simulink model "Sw_PMSMCtrl"  (R2025b)
settings: Solver=FixedStepDiscrete  StartTime=0.0  StopTime=10.0  RelTol=1e-3
values from neighbouring files (symbols this model uses):
  Par_Mdc_cboUdqCmd_Ovrd = 0    [Sw_PMSMCtrl.sldd]
  Par_Mdc_cfCurFc = 1000.0    [Sw_PMSMCtrl.sldd]
  Par_Mdc_cfKad = 1.0    [Sw_PMSMCtrl.sldd]
  Par_Mdc_cfKaq = 1.0    [Sw_PMSMCtrl.sldd]
  Par_Mdc_cfUdCmd = 0.0    [Sw_PMSMCtrl.sldd]
  Par_Mdc_cfUqCmd = 5.0    [Sw_PMSMCtrl.sldd]
  Par_Mtr_cfFlux = 0.0103693297    [Sw_PMSMCtrl.sldd]
  Par_Mtr_cfLd = 0.00085    [Sw_PMSMCtrl.sldd]
  Par_Mtr_cfLq = 0.00105    [Sw_PMSMCtrl.sldd]
  Par_Mtr_cfRs = 0.75    [Sw_PMSMCtrl.sldd]
  Par_Mtr_cuNp = 5    [Sw_PMSMCtrl.sldd]
  Par_Sw_cdTs = 5.0E-5    [Sw_PMSMCtrl.sldd]
libraries: Lib_PMSMCtrl x7, mcbeeMathTransformLib x3, Lib_General x2, mcbcontrolslib x1
settings Model: DataDictionary=Sw_PMSMCtrl.sldd  Creator=62555  LastModifiedBy=62555
settings SolverCC: MinimalZcImpactIntegration=on
settings OptimizationCC: DefaultParameterBehavior=Inlined  UseDivisionForNetSlopeComputation=on  GainParamInheritBuiltInType=on  UseFloatMulNetSlope=on  DefaultUnderspecifiedDataType=single  InlineInvariantSignals=on  PassReuseOutputArgsAs=Individual arguments  ZeroExternalMemoryAtStartup=off  ZeroInternalMemoryAtStartup=off  NoFixptDivByZeroProtection=on  EfficientFloat2IntCast=on  LifeSpan=1  MaxStackSize=64  OptimizeBlockOrder=speed  DifferentSizesBufferReuse=on  EfficientTunableParamExpr=on
settings DebuggingCC: SignalInfNanChecking=error  SignalRangeChecking=error  ReadBeforeWriteMsg=EnableAllAsError  WriteAfterWriteMsg=EnableAllAsError  WriteAfterReadMsg=EnableAllAsError  CheckMatrixSingularityMsg=error  IntegerOverflowMsg=error  ParameterPrecisionLossMsg=none  ParameterTunabilityLossMsg=error  UnconnectedInputMsg=error  UnconnectedOutputMsg=error  UnconnectedLineMsg=error  UniqueDataStoreMsg=error  AssertControl=DisableAll  SFUndirectedBroadcastEventsDiag=error  IntegerSaturationMsg=error  VariantConditionMismatch=error
settings HardwareCC: ProdBitPerPointer=32.0  ProdBitPerSizeT=32.0  ProdBitPerPtrDiffT=32.0  ProdLargestAtomicInteger=Long  ProdLargestAtomicFloat=Double  ProdWordSize=32.0  ProdLongLongMode=on  ProdHWDeviceType=ARM Compatible->ARM Cortex-M
settings ModelReferenceCC: UpdateModelReferenceTargets=IfOutOfDate  ModelReferenceNumInstancesAllowed=Single
settings SFSimCC: SFSimEcho=off  CompileTimeRecursionLimit=0.0  EnableRuntimeRecursion=off  MATLABDynamicMemAlloc=off
settings RTWCC: SystemTargetFile=ert.tlc  GenCodeOnly=on  TemplateMakefile=ert_default_tmf  GenerateReport=on  Toolchain=MinGW64 | gmake (64-bit Windows)  LaunchReport=on  GPUComputeCapability=3.5  Description=Embedded Coder
settings CodeAppCC: ForceParamTrailComments=on  IgnoreCustomStorageClasses=off  IgnoreTestpoints=on  OperatorAnnotations=on  SimulinkDataObjDesc=on  SFDataObjDesc=on  CustomSymbolStrGlobalVar=rt$N$M  CustomSymbolStrType=$N$M  CustomSymbolStrFcn=$N$M$F  CustomSymbolStrMacro=$N$M  InsertBlockDesc=on
settings ERTTargetCC: ExtModeTransport=3.0  ExtModeStaticAlloc=on  ExtModeStaticAllocSize=2048.0  ExtModeMexFile=ext_xcp  ExtModeIntrfLevel=Level2 - Open  ERTCustomFileTemplate=example_file_process.tlc  SuppressUnreachableDefaultCases=off  EnableSignedLeftShifts=off  EnableSignedRightShifts=off  DynamicArrayContainerType=coder::array  TargetLangStandard=C99 (ISO)  UtilityFuncGeneration=Shared location  IncludeMdlTerminateFcn=off  CombineSignalStateStructs=on  SupportAbsoluteTime=off  SubcomponentCodeInterfacePackaging=Nonreusable function  SupportComplex=off  SupportNonInlinedSFcns=on  ParenthesesLevel=Standards  CastingMode=Standards  GenerateSharedConstants=off

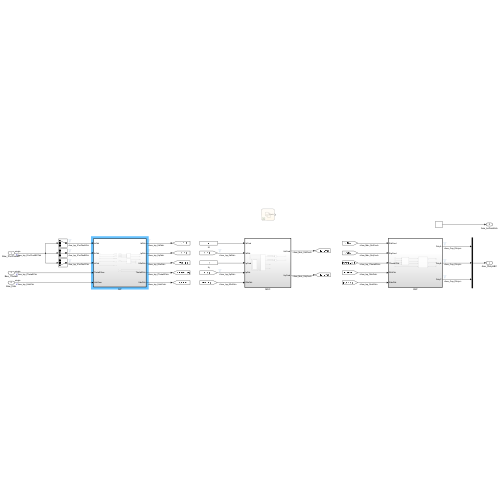
[thumbnail: Simulink's stored preview of the top-level diagram]
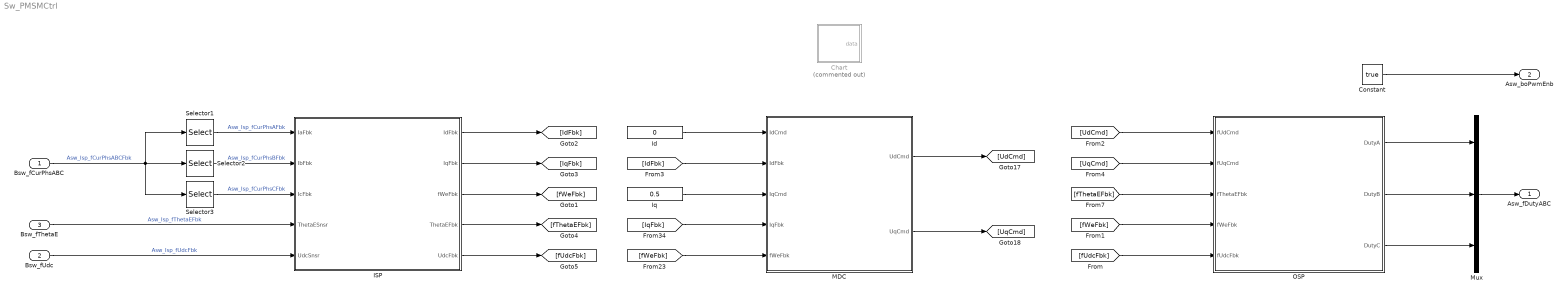
== system Sw_PMSMCtrl ==
  Bsw_fCurPhsABC : Inport  OutDataTypeStr=single  PortDimensions=3  SampleTime=Par_Sw_cdTs
  Bsw_fUdc : Inport  Port=2  OutDataTypeStr=single  SampleTime=Par_Sw_cdTs
  Bsw_fThetaE : Inport  Port=3  OutDataTypeStr=single  SampleTime=Par_Sw_cdTs
  Chart : Stateflow chart  Commented=on  TreatAsAtomicUnit=on
  Constant : Constant  Value=true  OutDataTypeStr=boolean  SampleTime=-1
  ISP : Subsystem  TreatAsAtomicUnit=on  RTWFileName=Asw_ISP
      settings: RTWSystemCode=Nonreusable function  RTWFcnNameOpts=Use subsystem name  RTWFileNameOpts=User specified  FunctionInterfaceSpec=Allow arguments (Optimized)
  Id : Constant  Value=0  OutDataTypeStr=single  SampleTime=-1
  Iq : Constant  Value=0.5  OutDataTypeStr=single  SampleTime=-1
  MDC : Subsystem  TreatAsAtomicUnit=on  RTWFileName=Asw_CLC
      settings: RTWSystemCode=Nonreusable function  RTWFcnNameOpts=Use subsystem name  RTWFileNameOpts=User specified  FunctionInterfaceSpec=Allow arguments (Optimized)
  Mux : Mux  Inputs=3
  OSP : Subsystem  TreatAsAtomicUnit=on  RTWFileName=Asw_Osp
      settings: RTWSystemCode=Nonreusable function  RTWFcnNameOpts=Use subsystem name  RTWFileNameOpts=User specified  FunctionInterfaceSpec=Allow arguments (Optimized)
  Selector1 : Selector  InputPortWidth=3  IndexOptions=Index vector (dialog)  Indices=[1]  OutputSizes=1
  Selector2 : Selector  InputPortWidth=3  IndexOptions=Index vector (dialog)  Indices=[2]  OutputSizes=1
  Selector3 : Selector  InputPortWidth=3  IndexOptions=Index vector (dialog)  Indices=[3]  OutputSizes=1
  Asw_fDutyABC : Outport
  Asw_boPwmEnb : Outport  Port=2
  wires:
  Selector1/1 -> ISP/1(IaFbk)  "Asw_Isp_fCurPhsAFbk"
  Selector2/1 -> ISP/2(IbFbk)  "Asw_Isp_fCurPhsBFbk"
  Selector3/1 -> ISP/3(IcFbk)  "Asw_Isp_fCurPhsCFbk"
  Bsw_fThetaE/1 -> ISP/4(ThetaESnsr)  "Asw_Isp_fThetaEFbk"
  Bsw_fUdc/1 -> ISP/5(UdcSnsr)  "Asw_Isp_fUdcFbk"
  ISP/1(IdFbk) -> [IdFbk]
  ISP/2(IqFbk) -> [IqFbk]
  ISP/3(fWeFbk) -> [fWeFbk]
  ISP/4(ThetaEFbk) -> [fThetaEFbk]
  ISP/5(UdcFbk) -> [fUdcFbk]
  Id/1 -> MDC/1(IdCmd)
  [IdFbk] -> MDC/2(IdFbk)
  Iq/1 -> MDC/3(IqCmd)
  [IqFbk] -> MDC/4(IqFbk)
  [fWeFbk] -> MDC/5(fWeFbk)
  MDC/1(UdCmd) -> [UdCmd]
  MDC/2(UqCmd) -> [UqCmd]
  [UdCmd] -> OSP/1(fUdCmd)
  [UqCmd] -> OSP/2(fUqCmd)
  [fThetaEFbk] -> OSP/3(fThetaEFbk)
  [fWeFbk] -> OSP/4(fWeFbk)
  [fUdcFbk] -> OSP/5(fUdcFbk)
  Constant/1 -> Asw_boPwmEnb/1
  OSP/1(DutyA) -> Mux/1
  OSP/2(DutyB) -> Mux/2
  OSP/3(DutyC) -> Mux/3
  Mux/1 -> Asw_fDutyABC/1
  Bsw_fCurPhsABC/1 -> Selector3/1, Selector2/1, Selector1/1  "Asw_Isp_fCurPhsABCFbk"

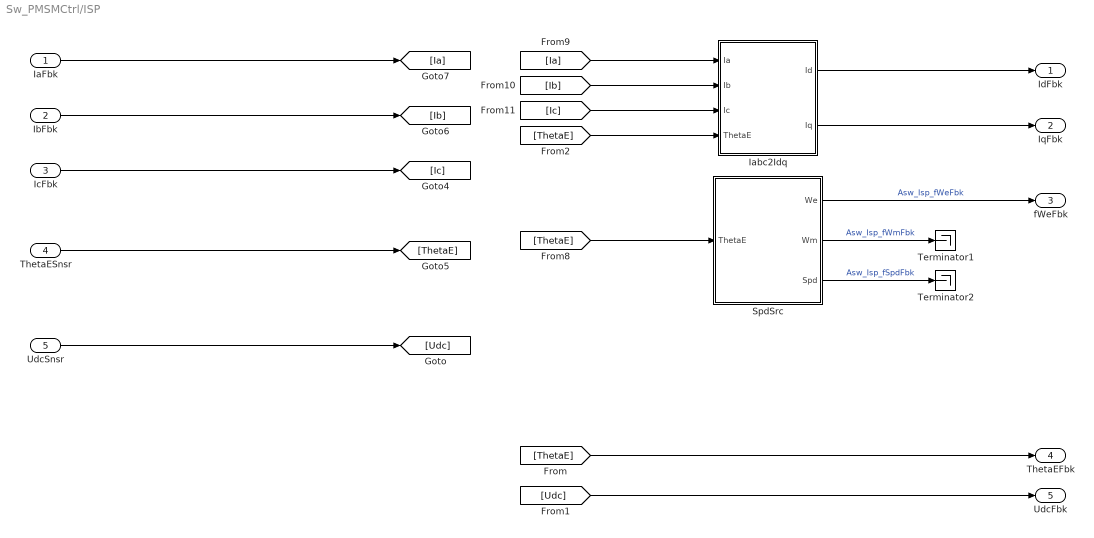
== system Sw_PMSMCtrl/ISP ==
  IaFbk : Inport
  IbFbk : Inport  Port=2
  IcFbk : Inport  Port=3
  ThetaESnsr : Inport  Port=4
  UdcSnsr : Inport  Port=5
  Iabc2Idq : Subsystem  TreatAsAtomicUnit=on
      settings: RTWSystemCode=Nonreusable function  RTWFcnNameOpts=Use subsystem name  FunctionInterfaceSpec=Allow arguments (Optimized)
  SpdSrc : Subsystem  TreatAsAtomicUnit=on
      settings: RTWSystemCode=Nonreusable function  RTWFcnNameOpts=Use subsystem name  FunctionInterfaceSpec=Allow arguments (Optimized)
  Terminator1 : Terminator
  Terminator2 : Terminator
  IdFbk : Outport
  IqFbk : Outport  Port=2
  fWeFbk : Outport  Port=3
  ThetaEFbk : Outport  Port=4
  UdcFbk : Outport  Port=5
  wires:
  SpdSrc/2(Wm) -> Terminator1/1  "Asw_Isp_fWmFbk"
  SpdSrc/3(Spd) -> Terminator2/1  "Asw_Isp_fSpdFbk"
  [ThetaE] -> Iabc2Idq/4(ThetaE)
  UdcSnsr/1 -> [Udc]
  [Ib] -> Iabc2Idq/2(Ib)
  Iabc2Idq/1(Id) -> IdFbk/1
  [ThetaE] -> SpdSrc/1(ThetaE)
  ThetaESnsr/1 -> [ThetaE]
  IcFbk/1 -> [Ic]
  IbFbk/1 -> [Ib]
  [Ia] -> Iabc2Idq/1(Ia)
  [Ic] -> Iabc2Idq/3(Ic)
  IaFbk/1 -> [Ia]
  SpdSrc/1(We) -> fWeFbk/1  "Asw_Isp_fWeFbk"
  Iabc2Idq/2(Iq) -> IqFbk/1
  [ThetaE] -> ThetaEFbk/1
  [Udc] -> UdcFbk/1

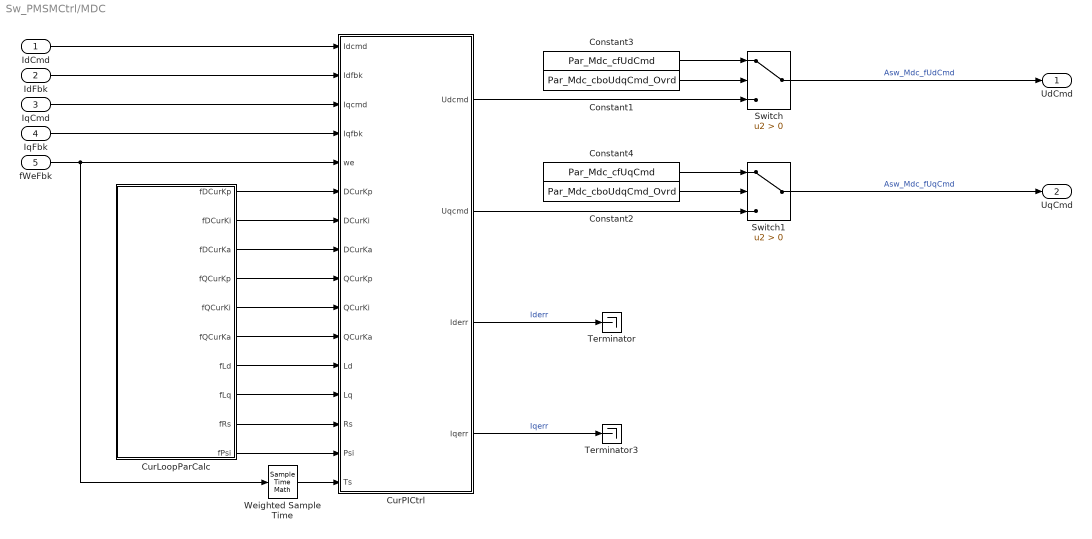
== system Sw_PMSMCtrl/MDC ==
  IdCmd : Inport
  IdFbk : Inport  Port=2
  IqCmd : Inport  Port=3
  IqFbk : Inport  Port=4
  fWeFbk : Inport  Port=5
  Constant1 : Constant  Value=Par_Mdc_cboUdqCmd_Ovrd  OutDataTypeStr=boolean  SampleTime=-1
  Constant2 : Constant  Value=Par_Mdc_cboUdqCmd_Ovrd  OutDataTypeStr=boolean  SampleTime=-1
  Constant3 : Constant  Value=Par_Mdc_cfUdCmd  OutDataTypeStr=single  SampleTime=-1
  Constant4 : Constant  Value=Par_Mdc_cfUqCmd  OutDataTypeStr=single  SampleTime=-1
  CurLoopParCalc : Subsystem
  CurPICtrl : MATLAB Function  TreatAsAtomicUnit=on
      settings: RTWSystemCode=Nonreusable function  RTWFcnNameOpts=Use subsystem name  FunctionInterfaceSpec=Allow arguments (Optimized)
  Switch : Switch  Criteria=u2 > Threshold  SaturateOnIntegerOverflow=off  InputSameDT=off
  Switch1 : Switch  Criteria=u2 > Threshold  SaturateOnIntegerOverflow=off  InputSameDT=off
  Terminator : Terminator
  Terminator3 : Terminator
  Weighted Sample Time : SampleTimeMath  TsampMathOp=Ts Only
  UdCmd : Outport
  UqCmd : Outport  Port=2
  wires:
  CurPICtrl/2(Uqcmd) -> Switch1/3
  CurPICtrl/3(Iderr) -> Terminator/1  "Iderr"
  IqCmd/1 -> CurPICtrl/3(Iqcmd)
  fWeFbk/1 -> Weighted Sample Time/1, CurPICtrl/5(we)
  IdCmd/1 -> CurPICtrl/1(Idcmd)
  CurPICtrl/1(Udcmd) -> Switch/3
  Weighted Sample Time/1 -> CurPICtrl/16(Ts)
  CurPICtrl/4(Iqerr) -> Terminator3/1  "Iqerr"
  IqFbk/1 -> CurPICtrl/4(Iqfbk)
  IdFbk/1 -> CurPICtrl/2(Idfbk)
  Constant2/1 -> Switch1/2
  Switch/1 -> UdCmd/1  "Asw_Mdc_fUdCmd"
  Constant4/1 -> Switch1/1
  Constant1/1 -> Switch/2
  Constant3/1 -> Switch/1
  Switch1/1 -> UqCmd/1  "Asw_Mdc_fUqCmd"
  CurLoopParCalc/1(fDCurKp) -> CurPICtrl/6(DCurKp)
  CurLoopParCalc/2(fDCurKi) -> CurPICtrl/7(DCurKi)
  CurLoopParCalc/3(fDCurKa) -> CurPICtrl/8(DCurKa)
  CurLoopParCalc/4(fQCurKp) -> CurPICtrl/9(QCurKp)
  CurLoopParCalc/5(fQCurKi) -> CurPICtrl/10(QCurKi)
  CurLoopParCalc/6(fQCurKa) -> CurPICtrl/11(QCurKa)
  CurLoopParCalc/7(fLd) -> CurPICtrl/12(Ld)
  CurLoopParCalc/8(fLq) -> CurPICtrl/13(Lq)
  CurLoopParCalc/9(fRs) -> CurPICtrl/14(Rs)
  CurLoopParCalc/10(fPsi) -> CurPICtrl/15(Psi)

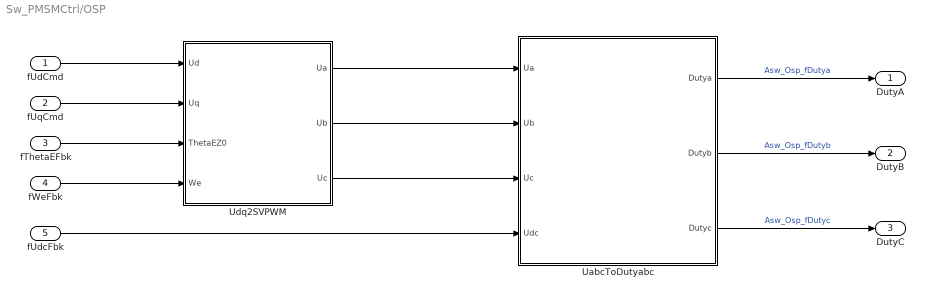
== system Sw_PMSMCtrl/OSP ==
  fUdCmd : Inport
  fUqCmd : Inport  Port=2
  fThetaEFbk : Inport  Port=3
  fWeFbk : Inport  Port=4
  fUdcFbk : Inport  Port=5
  UabcToDutyabc : Subsystem  TreatAsAtomicUnit=on
      settings: RTWSystemCode=Nonreusable function  RTWFcnNameOpts=Use subsystem name  FunctionInterfaceSpec=Allow arguments (Optimized)
  Udq2SVPWM : Subsystem  TreatAsAtomicUnit=on
      settings: RTWSystemCode=Nonreusable function  RTWFcnNameOpts=Use subsystem name  FunctionInterfaceSpec=Allow arguments (Optimized)
  DutyA : Outport
  DutyB : Outport  Port=2
  DutyC : Outport  Port=3
  wires:
  fThetaEFbk/1 -> Udq2SVPWM/3(ThetaEZ0)
  Udq2SVPWM/1(Ua) -> UabcToDutyabc/1(Ua)
  Udq2SVPWM/2(Ub) -> UabcToDutyabc/2(Ub)
  fUdCmd/1 -> Udq2SVPWM/1(Ud)
  fUdcFbk/1 -> UabcToDutyabc/4(Udc)
  Udq2SVPWM/3(Uc) -> UabcToDutyabc/3(Uc)
  fUqCmd/1 -> Udq2SVPWM/2(Uq)
  fWeFbk/1 -> Udq2SVPWM/4(We)
  UabcToDutyabc/1(Dutya) -> DutyA/1  "Asw_Osp_fDutya"
  UabcToDutyabc/2(Dutyb) -> DutyB/1  "Asw_Osp_fDutyb"
  UabcToDutyabc/3(Dutyc) -> DutyC/1  "Asw_Osp_fDutyc"

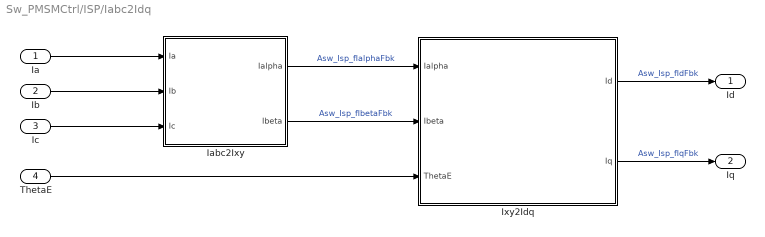
== system Sw_PMSMCtrl/ISP/Iabc2Idq ==
  Ia : Inport
  Ib : Inport  Port=2
  Ic : Inport  Port=3
  ThetaE : Inport  Port=4
  Iabc2Ixy : Subsystem  TreatAsAtomicUnit=on
      settings: RTWSystemCode=Nonreusable function  RTWFcnNameOpts=Use subsystem name  FunctionInterfaceSpec=Allow arguments (Optimized)
  Ixy2Idq : Subsystem  TreatAsAtomicUnit=on
      settings: RTWSystemCode=Nonreusable function  RTWFcnNameOpts=Use subsystem name  FunctionInterfaceSpec=Allow arguments (Optimized)
  Id : Outport
  Iq : Outport  Port=2
  wires:
  Ixy2Idq/2(Iq) -> Iq/1  "Asw_Isp_fIqFbk"
  Ia/1 -> Iabc2Ixy/1(Ia)
  ThetaE/1 -> Ixy2Idq/3(ThetaE)
  Ic/1 -> Iabc2Ixy/3(Ic)
  Ixy2Idq/1(Id) -> Id/1  "Asw_Isp_fIdFbk"
  Ib/1 -> Iabc2Ixy/2(Ib)
  Iabc2Ixy/2(Ibeta) -> Ixy2Idq/2(Ibeta)  "Asw_Isp_fIbetaFbk"
  Iabc2Ixy/1(Ialpha) -> Ixy2Idq/1(Ialpha)  "Asw_Isp_fIalphaFbk"

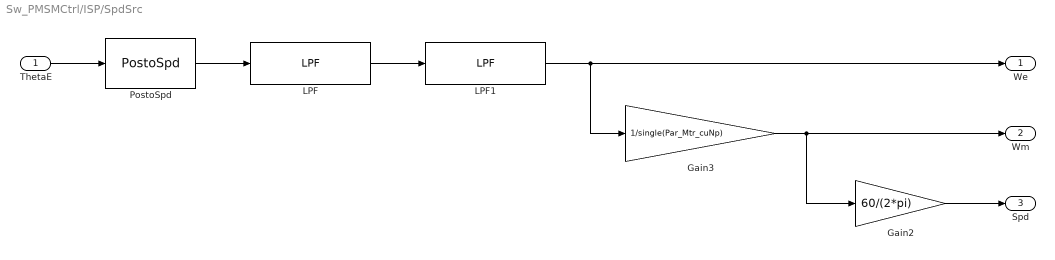
== system Sw_PMSMCtrl/ISP/SpdSrc ==
  ThetaE : Inport
  Gain2 : Gain  Gain=60/(2*pi)
  Gain3 : Gain  Gain=1/single(Par_Mtr_cuNp)
  LPF : Lib_General/LPF  fc=1e3  Initial_condition=0  ModType=Tustin
      settings: SourceProductName=Lib_General
      settings: AttributesFormatString=|
      | fc = %<fc>
      | DisMod = %<ModType>
  LPF1 : Lib_General/LPF  fc=1e3  Initial_condition=0  ModType=Tustin
      settings: SourceProductName=Lib_General
      settings: AttributesFormatString=|
      | fc = %<fc>
      | DisMod = %<ModType>
  PostoSpd : Lib_PMSMCtrl/PostoSpd
      settings: SourceProductName=Lib_PMSMCtrl
  We : Outport
  Wm : Outport  Port=2
  Spd : Outport  Port=3
  wires:
  PostoSpd/1 -> LPF/1
  ThetaE/1 -> PostoSpd/1
  Gain2/1 -> Spd/1
  Gain3/1 -> Gain2/1, Wm/1
  LPF/1 -> LPF1/1
  LPF1/1 -> We/1, Gain3/1

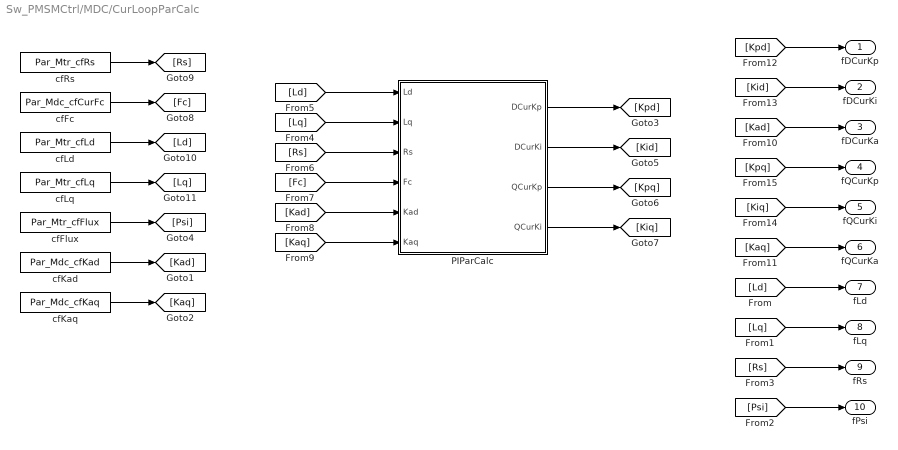
== system Sw_PMSMCtrl/MDC/CurLoopParCalc ==
  PIParCalc : MATLAB Function  TreatAsAtomicUnit=on
      settings: RTWSystemCode=Nonreusable function  RTWFcnNameOpts=Use subsystem name  FunctionInterfaceSpec=Allow arguments (Optimized)
  cfFc : Constant  Value=Par_Mdc_cfCurFc  OutDataTypeStr=single  SampleTime=-1
  cfFlux : Constant  Value=Par_Mtr_cfFlux  OutDataTypeStr=single  SampleTime=-1
  cfKad : Constant  Value=Par_Mdc_cfKad  OutDataTypeStr=single  SampleTime=-1
  cfKaq : Constant  Value=Par_Mdc_cfKaq  OutDataTypeStr=single  SampleTime=-1
  cfLd : Constant  Value=Par_Mtr_cfLd  OutDataTypeStr=single  SampleTime=-1
  cfLq : Constant  Value=Par_Mtr_cfLq  OutDataTypeStr=single  SampleTime=-1
  cfRs : Constant  Value=Par_Mtr_cfRs  OutDataTypeStr=single  SampleTime=-1
  fDCurKp : Outport
  fDCurKi : Outport  Port=2
  fDCurKa : Outport  Port=3
  fQCurKp : Outport  Port=4
  fQCurKi : Outport  Port=5
  fQCurKa : Outport  Port=6
  fLd : Outport  Port=7
  fLq : Outport  Port=8
  fRs : Outport  Port=9
  fPsi : Outport  Port=10
  wires:
  cfLq/1 -> [Lq]
  cfLd/1 -> [Ld]
  cfRs/1 -> [Rs]
  cfFc/1 -> [Fc]
  cfFlux/1 -> [Psi]
  [Ld] -> fLd/1
  [Lq] -> fLq/1
  [Psi] -> fPsi/1
  [Rs] -> fRs/1
  [Lq] -> PIParCalc/2(Lq)
  [Ld] -> PIParCalc/1(Ld)
  [Rs] -> PIParCalc/3(Rs)
  [Fc] -> PIParCalc/4(Fc)
  PIParCalc/1(DCurKp) -> [Kpd]
  cfKaq/1 -> [Kaq]
  cfKad/1 -> [Kad]
  [Kad] -> PIParCalc/5(Kad)
  [Kaq] -> PIParCalc/6(Kaq)
  [Kaq] -> fQCurKa/1
  [Kad] -> fDCurKa/1
  [Kpd] -> fDCurKp/1
  PIParCalc/2(DCurKi) -> [Kid]
  PIParCalc/3(QCurKp) -> [Kpq]
  PIParCalc/4(QCurKi) -> [Kiq]
  [Kid] -> fDCurKi/1
  [Kiq] -> fQCurKi/1
  [Kpq] -> fQCurKp/1

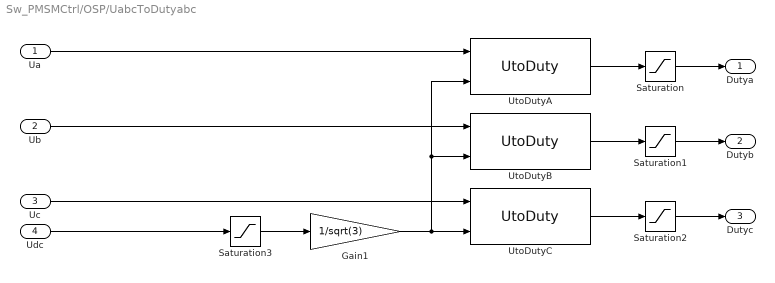
== system Sw_PMSMCtrl/OSP/UabcToDutyabc ==
  Ua : Inport
  Ub : Inport  Port=2
  Uc : Inport  Port=3
  Udc : Inport  Port=4
  Gain1 : Gain  Gain=1/sqrt(3)
  Saturation : Saturate  UpperLimit=single(1)  LowerLimit=single(0)
  Saturation1 : Saturate  UpperLimit=single(1)  LowerLimit=single(0)
  Saturation2 : Saturate  UpperLimit=single(1)  LowerLimit=single(0)
  Saturation3 : Saturate  UpperLimit=inf  LowerLimit=single(0.01)
  UtoDutyA : Lib_PMSMCtrl/UtoDuty
      settings: SourceProductName=Lib_PMSMCtrl
  UtoDutyB : Lib_PMSMCtrl/UtoDuty
      settings: SourceProductName=Lib_PMSMCtrl
  UtoDutyC : Lib_PMSMCtrl/UtoDuty
      settings: SourceProductName=Lib_PMSMCtrl
  Dutya : Outport
  Dutyb : Outport  Port=2
  Dutyc : Outport  Port=3
  wires:
  Uc/1 -> UtoDutyC/1
  Ub/1 -> UtoDutyB/1
  UtoDutyA/1 -> Saturation/1
  UtoDutyC/1 -> Saturation2/1
  UtoDutyB/1 -> Saturation1/1
  Ua/1 -> UtoDutyA/1
  Udc/1 -> Saturation3/1
  Saturation3/1 -> Gain1/1
  Gain1/1 -> UtoDutyA/2, UtoDutyB/2, UtoDutyC/2
  Saturation/1 -> Dutya/1
  Saturation1/1 -> Dutyb/1
  Saturation2/1 -> Dutyc/1

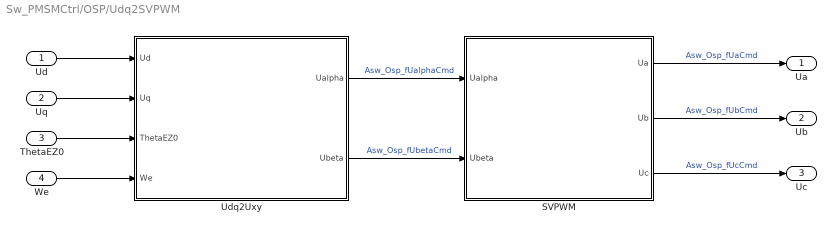
== system Sw_PMSMCtrl/OSP/Udq2SVPWM ==
  Ud : Inport
  Uq : Inport  Port=2
  ThetaEZ0 : Inport  Port=3
  We : Inport  Port=4
  SVPWM : Subsystem  TreatAsAtomicUnit=on
      settings: RTWSystemCode=Nonreusable function  RTWFcnNameOpts=Use subsystem name  FunctionInterfaceSpec=Allow arguments (Optimized)
  Udq2Uxy : Subsystem  TreatAsAtomicUnit=on
      settings: RTWSystemCode=Nonreusable function  RTWFcnNameOpts=Use subsystem name  FunctionInterfaceSpec=Allow arguments (Optimized)
  Ua : Outport
  Ub : Outport  Port=2
  Uc : Outport  Port=3
  wires:
  Ud/1 -> Udq2Uxy/1(Ud)
  Udq2Uxy/1(Ualpha) -> SVPWM/1(Ualpha)  "Asw_Osp_fUalphaCmd"
  ThetaEZ0/1 -> Udq2Uxy/3(ThetaEZ0)
  We/1 -> Udq2Uxy/4(We)
  Uq/1 -> Udq2Uxy/2(Uq)
  Udq2Uxy/2(Ubeta) -> SVPWM/2(Ubeta)  "Asw_Osp_fUbetaCmd"
  SVPWM/3(Uc) -> Uc/1  "Asw_Osp_fUcCmd"
  SVPWM/1(Ua) -> Ua/1  "Asw_Osp_fUaCmd"
  SVPWM/2(Ub) -> Ub/1  "Asw_Osp_fUbCmd"

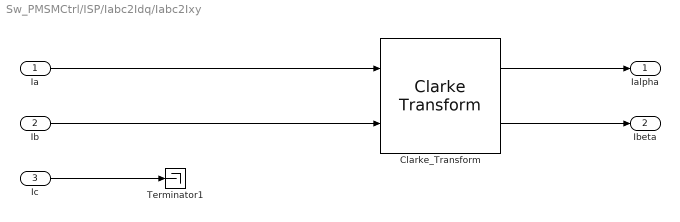
== system Sw_PMSMCtrl/ISP/Iabc2Idq/Iabc2Ixy ==
  Ia : Inport
  Ib : Inport  Port=2
  Ic : Inport  Port=3
  Clarke_Transform : mcbeeMathTransformLib/Clarke Transform  VariantControl=Variant2  PowerInvariant=off  UseWithEmbedded=on  PhaseInput=Two inputs
  Terminator1 : Terminator
  Ialpha : Outport
  Ibeta : Outport  Port=2
  wires:
  Ib/1 -> Clarke_Transform/2
  Ia/1 -> Clarke_Transform/1
  Clarke_Transform/2 -> Ibeta/1
  Clarke_Transform/1 -> Ialpha/1
  Ic/1 -> Terminator1/1

== system Sw_PMSMCtrl/ISP/Iabc2Idq/Ixy2Idq ==
  Ialpha : Inport
  Ibeta : Inport  Port=2
  ThetaE : Inport  Port=3
  Park_Transform : mcbeeMathTransformLib/Clarke to Park Angle Transform  AxisAlignment=D-axis  UseWithEmbedded=on  PhaseInput=Two inputs  ThetaInput=Sine and Cosine electrical position  AngleInput=Per-unit  N_points=1024
  SinCos_Calc : Lib_PMSMCtrl/SinCos_Calc
      settings: SourceProductName=Lib_PMSMCtrl
  Id : Outport
  Iq : Outport  Port=2
  wires:
  Ibeta/1 -> Park_Transform/2
  ThetaE/1 -> SinCos_Calc/1
  SinCos_Calc/2 -> Park_Transform/4
  Park_Transform/1 -> Id/1
  SinCos_Calc/1 -> Park_Transform/3
  Park_Transform/2 -> Iq/1
  Ialpha/1 -> Park_Transform/1

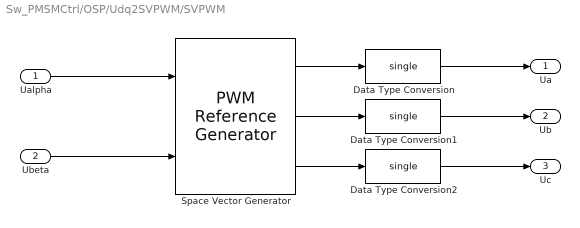
== system Sw_PMSMCtrl/OSP/Udq2SVPWM/SVPWM ==
  Ualpha : Inport
  Ubeta : Inport  Port=2
  Data Type Conversion : DataTypeConversion  OutDataTypeStr=single  SaturateOnIntegerOverflow=off  RndMeth=Floor
  Data Type Conversion1 : DataTypeConversion  OutDataTypeStr=single  SaturateOnIntegerOverflow=off  RndMeth=Floor
  Data Type Conversion2 : DataTypeConversion  OutDataTypeStr=single  SaturateOnIntegerOverflow=off  RndMeth=Floor
  Space Vector Generator : mcbcontrolslib/PWM Reference Generator  inSignal=Valphabeta  modType=SVM: space vector modulation
  Ua : Outport
  Ub : Outport  Port=2
  Uc : Outport  Port=3
  wires:
  Data Type Conversion2/1 -> Uc/1
  Space Vector Generator/1 -> Data Type Conversion/1
  Space Vector Generator/2 -> Data Type Conversion1/1
  Data Type Conversion/1 -> Ua/1
  Space Vector Generator/3 -> Data Type Conversion2/1
  Data Type Conversion1/1 -> Ub/1
  Ubeta/1 -> Space Vector Generator/2
  Ualpha/1 -> Space Vector Generator/1

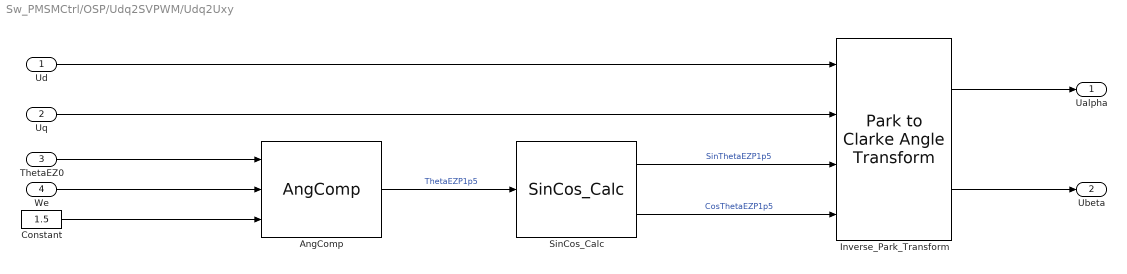
== system Sw_PMSMCtrl/OSP/Udq2SVPWM/Udq2Uxy ==
  Ud : Inport
  Uq : Inport  Port=2
  ThetaEZ0 : Inport  Port=3
  We : Inport  Port=4
  AngComp : Lib_PMSMCtrl/AngComp
      settings: SourceProductName=Lib_PMSMCtrl
  Constant : Constant  Value=1.5  OutDataTypeStr=single  SampleTime=-1
  Inverse_Park_Transform : mcbeeMathTransformLib/Park to Clarke Angle Transform  AxisAlignment=D-axis  UseWithEmbedded=on  PhaseInput=Two inputs  ThetaInput=Sine and Cosine electrical position  AngleInput=Per-unit  N_points=1024
  SinCos_Calc : Lib_PMSMCtrl/SinCos_Calc
      settings: SourceProductName=Lib_PMSMCtrl
  Ualpha : Outport
  Ubeta : Outport  Port=2
  wires:
  ThetaEZ0/1 -> AngComp/1
  Uq/1 -> Inverse_Park_Transform/2
  Inverse_Park_Transform/1 -> Ualpha/1
  AngComp/1 -> SinCos_Calc/1  "ThetaEZP1p5"
  SinCos_Calc/1 -> Inverse_Park_Transform/3  "SinThetaEZP1p5"
  SinCos_Calc/2 -> Inverse_Park_Transform/4  "CosThetaEZP1p5"
  Inverse_Park_Transform/2 -> Ubeta/1
  Constant/1 -> AngComp/3
  Ud/1 -> Inverse_Park_Transform/1
  We/1 -> AngComp/2

== matlab function Sw_PMSMCtrl/MDC/CurLoopParCalc/PIParCalc ==
  data: Ld input; DCurKp output; DCurKi output; QCurKp output; QCurKi output; Lq input; Rs input; Fc input; Kad input; Kaq input
function [DCurKp, DCurKi, QCurKp, QCurKi] = PIParCalc(Ld, Lq, Rs, Fc, Kad, Kaq)

  Wc = Fc * 2 * single(pi);

  DCurKp = Ld * Wc;
  DCurKi = Rs * (1 + Kad * single(1)) * Wc;

  QCurKp = Lq * Wc;
  QCurKi = Rs * (1 + Kaq * single(1)) * Wc;
end

== matlab function Sw_PMSMCtrl/MDC/CurPICtrl ==
  data: Idcmd input; Udcmd output; Uqcmd output; Idfbk input; Iqcmd input; Iqfbk input; we input; DCurKp input; DCurKi input; DCurKa input; QCurKp input; QCurKi input; QCurKa input; Ld input; Lq input; Rs input; Psi input; Ts input; Iderr output; Iqerr output
function [Udcmd, Uqcmd, Iderr, Iqerr] = CurPICtrl(Idcmd, Idfbk, Iqcmd, Iqfbk, we, DCurKp, DCurKi, DCurKa, QCurKp, QCurKi, QCurKa, Ld, Lq, Rs, Psi, Ts)
  
  persistent Dui;
  persistent Qui;

  if isempty(Dui)
    Dui = single(0);
    Qui = single(0);
  end
  
  % d轴PI控制
  Iderr = Idcmd - Idfbk;
  Dup = DCurKp * Iderr;
  Dui = Dui + DCurKi * Iderr * Ts;
  UdPI = Dup + Dui;
  
  % d轴主动阻尼
  UdActDamp = -DCurKa * Rs * Idfbk;
  
  % d轴电压合成
  Udcmd = UdPI + UdActDamp - we * Lq * Iqfbk;
  
  % q轴PI控制
  Iqerr = Iqcmd - Iqfbk;
  Qup = QCurKp * Iqerr;
  Qui = Qui + QCurKi * Iqerr * Ts;
  UqPI = Qup + Qui;
  
  % q轴主动阻尼
  UqActDamp = -QCurKa * Rs * Iqfbk;
  
  % q轴电压合成
  Uqcmd = UqPI + UqActDamp + we * Ld *Idfbk + we * Psi;

end

== stateflow chart Sw_PMSMCtrl/Chart ==
  data: data output double
